simulink model "sistema4"  (R2026b)
settings: Solver=ode15s  MaxStep=1e-2
libraries: fl_lib x14, nesl_utility x6, slpidlib x1
settings Model: Creator=Admin  LastModifiedBy=nicol
settings DataIOCC: DSMLogging=off  ReturnWorkspaceOutputs=off  SaveOutput=off  SignalLogging=off  TimeSaveName=t
settings DebuggingCC: AlgebraicLoopMsg=none  ArtificialAlgebraicLoopMsg=none  MaxConsecutiveZCsMsg=none
settings RTWCC: GPUComputeCapability=5.0
settings SimscapeCC: SimscapeLogType=all  SimscapeNominalValues="[{\"value\":\"1\",\"unit\":\"A\"},{\"value\":\"1\",\"unit\":\"bar\"},{\"value\":\"1\",\"unit\":\"cm^2\"},{\"value\":\"1\",\"unit\":\"cm^3/s\"},{\"value\":\"1\",\"unit\":\"kJ/kg\"},{\"value\":\"1\",\"unit\":\"kW\"},{\"value\":\"1\",\"unit\":\"l\"},{\"value\":\"1\",\"unit\":\"N\"},{\"value\":\"1\",\"unit\":\"N*m\"},{\"value\":\"1\",\"unit\":\"V\"},{\"value\":\"0.001\",\"unit\":\"Wb\"}]"  SimscapeUseEnergyAccounting=off

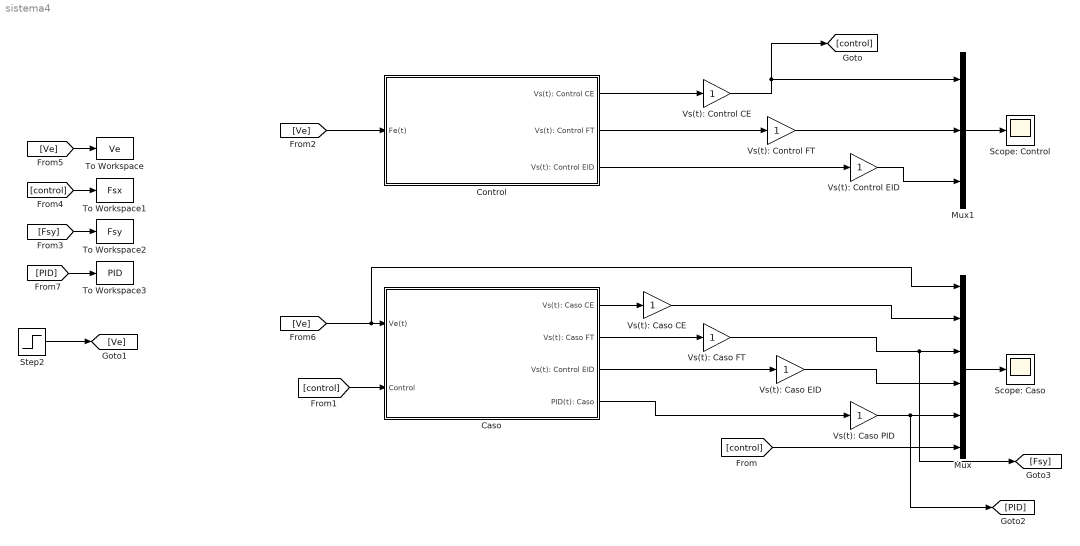
== system sistema4 ==
  Caso : Subsystem
  Control : Subsystem
  Mux : Mux  Inputs=6
  Mux1 : Mux  Inputs=3
  Scope: Caso : Scope
      settings: ActiveDisplayYMinimum=-0.12376521739333951  ActiveDisplayYMaximum=1.1138869565400558
  Scope: Control : Scope
      settings: ActiveDisplayYMinimum=-0.12376521739412114  ActiveDisplayYMaximum=1.1138869565470904
  Step2 : Step  Time=0  SampleTime=0
  To Workspace : ToWorkspace  VariableName=Ve  SampleTime=-1
  To Workspace1 : ToWorkspace  VariableName=Fsx  SampleTime=-1
  To Workspace2 : ToWorkspace  VariableName=Fsy  SampleTime=-1
  To Workspace3 : ToWorkspace  VariableName=PID  SampleTime=-1
  Vs(t): Caso CE : Gain
  Vs(t): Caso EID : Gain
  Vs(t): Caso FT : Gain
  Vs(t): Caso PID : Gain
  Vs(t): Control CE : Gain
  Vs(t): Control EID : Gain
  Vs(t): Control FT : Gain
  wires:
  Caso/2(Vs(t): Caso FT) -> Vs(t): Caso FT/1
  Caso/3(Vs(t): Control EID) -> Vs(t): Caso EID/1
  Vs(t): Caso EID/1 -> Mux/4
  Mux/1 -> Scope: Caso/1
  Mux1/1 -> Scope: Control/1
  Control/1(Vs(t): Control CE) -> Vs(t): Control CE/1
  [Ve] -> Control/1(Fe(t))
  [Ve] -> Mux/1, Caso/1(Ve(t))
  Control/3(Vs(t): Control EID) -> Vs(t): Control EID/1
  Vs(t): Control EID/1 -> Mux1/3
  Vs(t): Control FT/1 -> Mux1/2
  Control/2(Vs(t): Control FT) -> Vs(t): Control FT/1
  Caso/1(Vs(t): Caso CE) -> Vs(t): Caso CE/1
  Vs(t): Control CE/1 -> [control], Mux1/1
  Vs(t): Caso CE/1 -> Mux/2
  Vs(t): Caso FT/1 -> Mux/3, [Fsy]
  Caso/4(PID(t): Caso) -> Vs(t): Caso PID/1
  Vs(t): Caso PID/1 -> [PID], Mux/5
  [control] -> Mux/6
  [control] -> Caso/2(Control)
  [Fsy] -> To Workspace2/1
  [control] -> To Workspace1/1
  [PID] -> To Workspace3/1
  [Ve] -> To Workspace/1
  Step2/1 -> [Ve]

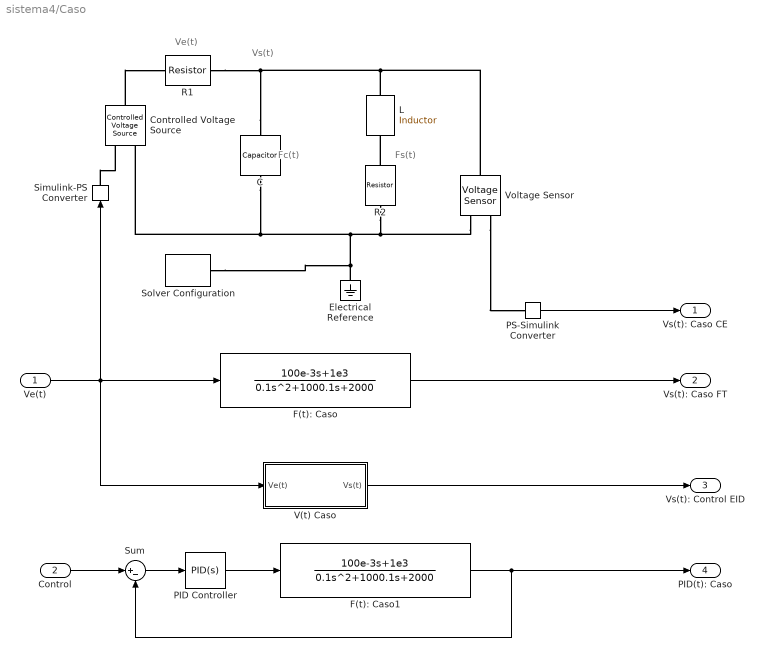
== system sistema4/Caso ==
  note: Ve(t)
  note: Vs(t)
  note: Fc(t)
  note: Fs(t)
  Ve(t) : Inport
  Control : Inport  Port=2
  C : fl_lib/Electrical/Electrical Elements/Capacitor  c=1000 uF  r=1e-6 Ohm  g=0 1/Ohm  i_specify=off  i_priority=None  i=0 A  i_nominal_specify=off  i_nominal_value=1  i_nominal_unit=A  v_specify=off  v_priority=None  v=0 V  v_nominal_specify=off  v_nominal_value=1  v_nominal_unit=V  vc_specify=off  vc_priority=High  vc=0 V  vc_nominal_specify=off  vc_nominal_value=1  vc_nominal_unit=V
  Controlled Voltage Source : fl_lib/Electrical/Electrical Sources/Controlled Voltage Source
  Electrical Reference : fl_lib/Electrical/Electrical Elements/Electrical Reference
  F(t): Caso : TransferFcn  Numerator=[100e-3 1e3]  Denominator=[0.1 1000.1 2000]
  F(t): Caso1 : TransferFcn  Numerator=[100e-3 1e3]  Denominator=[0.1 1000.1 2000]
  L : fl_lib/Electrical/Electrical Elements/Inductor  l=100e-3 H  r=0 Ohm  g=1e-9 1/Ohm  i_specify=off  i_priority=None  i=0 A  i_nominal_specify=off  i_nominal_value=1  i_nominal_unit=A  v_specify=off  v_priority=None  v=0 V  v_nominal_specify=off  v_nominal_value=1  v_nominal_unit=V  i_L_specify=off  i_L_priority=High  i_L=0 A  i_L_nominal_specify=off  i_L_nominal_value=1  i_L_nominal_unit=A
  PID Controller : slpidlib/PID Controller  Controller=PID  Form=Parallel  TimeDomain=Continuous-time  UseExternalTs=off  SampleTime=-1  IntegratorMethod=Forward Euler  FilterMethod=Forward Euler  ControllerParametersSource=internal  P=1315.96113707451  I=320705.002123674  UseKiTs=off  D=0.179701213263049  UseExternalDerivativeSource=off  N=5030.10216106345  UseFilter=on  TunerSelectOption=Transfer Function Based (PID Tuner App)  InitialConditionSource=internal  InitialConditionForIntegrator=0  InitialConditionForFilter=0  DifferentiatorICPrevScaledInput=0  ExternalReset=none  TrackingMode=off  Kt=1  LimitOutput=off  SatLimitsSource=internal  UpperSaturationLimit=inf  LowerSaturationLimit=-inf  LinearizeAsGain=on  AntiWindupMode=none  Kb=1  LimitIntegrator=off  UpperIntegratorSaturationLimit=inf  LowerIntegratorSaturationLimit=-inf  POutMin=[]  POutMax=[]  IOutMin=[]  IOutMax=[]  DOutMin=[]  DOutMax=[]  NOutMin=[]  NOutMax=[]  SumOutMin=[]  SumOutMax=[]  SaturationOutMin=[]  SaturationOutMax=[]  PParamMin=[]  PParamMax=[]  IParamMin=[]  IParamMax=[]  DParamMin=[]  DParamMax=[]  NParamMin=[]  NParamMax=[]  KbParamMin=[]  KbParamMax=[]  KtParamMin=[]  KtParamMax=[]  KbOutMin=[]  KbOutMax=[]  KtOutMin=[]  KtOutMax=[]  IntegratorOutMin=[]  IntegratorOutMax=[]  FilterOutMin=[]  FilterOutMax=[]  SumI1OutMin=[]  SumI1OutMax=[]  SumI2OutMin=[]  SumI2OutMax=[]  SumI3OutMin=[]  SumI3OutMax=[]  SumI4OutMin=[]  SumI4OutMax=[]  SumDOutMin=[]  SumDOutMax=[]  DifferentiatorOutMin=[]  DifferentiatorOutMax=[]  FilterDiffOutCoefMin=[]  FilterDiffOutCoefMax=[]  ReciprocalOutMin=[]  ReciprocalOutMax=[]  SumDenOutMin=[]  SumDenOutMax=[]  SumNumOutMin=[]  SumNumOutMax=[]  DivideOutMin=[]  DivideOutMax=[]  UdiffTsProdOutMin=[]  UdiffTsProdOutMax=[]  NTsProdOutMin=[]  NTsProdOutMax=[]  UintegralTsProdOutMin=[]  UintegralTsProdOutMax=[]  UngainTsProdOutMin=[]  UngainTsProdOutMax=[]  ClampingZeroOutDataTypeStr=Inherit: Inherit via back propagation  ClampingZeroOutMin=[]  ClampingZeroOutMax=[]  FilterDenConstantOutDataTypeStr=Inherit: Inherit via back propagation  FilterDenConstantOutMin=[]  FilterDenConstantOutMax=[]  PCopyOutDataTypeStr=Inherit: Inherit via back propagation  PCopyOutMin=[]  PCopyOutMax=[]  NCopyOutDataTypeStr=Inherit: Inherit via back propagation  NCopyOutMin=[]  NCopyOutMax=[]  IntegratorContinuousStateAttributes=''  IntegratorStateMustResolveToSignalObject=off  IntegratorRTWStateStorageClass=Auto  FilterContinuousStateAttributes=''  FilterStateMustResolveToSignalObject=off  FilterRTWStateStorageClass=Auto  ParallelPVariant=InternalParameters  IdealPVariant=Disabled  IVariant=InternalParameters  DVariant=InternalParameters  IntegratorVariant=Continuous  SatVariant=Disabled  AWVariant=Passthrough  PCopyVariant=Disabled  TRVariant=Disabled  FdbkBlocksVariant=Forward  IdealPFdbkVariant=Disabled  SatFdbkVariant=Disabled  DerivativeFilterVariant=ContFilter  NVariant=InternalParameters  NCopyVariant=Disabled  FilterICVariant=InternalICsFilter  IntegratorICVariant=InternalICs  ExternalResetVariant=Disabled  TRSumVariant=Passthrough  SumFdbkVariant=Disabled  SumVariant=Sum_PID  TsampFilterVariant=InternalTs  TsampNgainVariant=Passthrough  TsampIntegralVariant=Disabled_SignalSpec  ExternalSaturationOutDataTypeStr=Inherit: Same as second input  DerivativeSourceVariant=ErrorSignal  PreIntVariant=InternalPreInt
  PS-Simulink Converter : nesl_utility/PS-Simulink Converter  PhysicalDomain=network_engine_domain  SubClassName=ps_output  LeftPortType=input  RightPortType=output  PseudoPeriodic=off  Frequencies=[]  VectorFormat=inherit  Unit=inherit  AffineConversion=off
  R1 : fl_lib/Electrical/Electrical Elements/Resistor  R=1 kOhm  i_specify=off  i_priority=None  i=0 A  i_nominal_specify=off  i_nominal_value=1  i_nominal_unit=A  v_specify=off  v_priority=None  v=0 V  v_nominal_specify=off  v_nominal_value=1  v_nominal_unit=V
  R2 : fl_lib/Electrical/Electrical Elements/Resistor  R=1 kOhm  i_specify=off  i_priority=None  i=0 A  i_nominal_specify=off  i_nominal_value=1  i_nominal_unit=A  v_specify=off  v_priority=None  v=0 V  v_nominal_specify=off  v_nominal_value=1  v_nominal_unit=V
  Simulink-PS Converter : nesl_utility/Simulink-PS Converter  PhysicalDomain=network_engine_domain  SubClassName=ps_input  LeftPortType=input  RightPortType=output  PseudoPeriodic=off  Frequencies=[]  NoiseDistribution=none  NoiseParameters=[]  Unit=1  AffineConversion=off  FilteringAndDerivatives=provide  SimscapeFilterOrder=1  InputFilterTimeConstant=0.001  UdotUserProvided=0
  Solver Configuration : nesl_utility/Solver Configuration  PhysicalDomain=network_engine_domain  SubClassName=solver  LeftPortType=input  RightPortType=generic  Tones=[]  Harmonics=[]  SimulateNoise=off  Profile=off  UseLocalSampling=off  EnableSwitchedLinearOptims=on  FrequencyDomain=off  UseCCode=off  RelTol=0.001  AbsTol=0.001  MinStep=1e-09  ToWorkspace=off  RevertToSquareIcSolve=off  NumHomotopyIterations=100  PhasorMode=off  PhasorModeNumHarmonics=1  ConsistencySolver=NEWTON_XTOL_AFTER_FTOL  CanonicalOrdering=UNORDERED  OptimizeIntermediates=UNOPTIMIZED  MulticoreSolverChoice=BACKWARD_EULER  IndexReductionMethod=DerivativeReplacement  DoDC=off  ResidualTolerance=1e-09  ConsistencyTolSource=GLOBAL  ConsistencyAbsTol=0.001  ConsistencyRelTol=0.001  ConsistencyTolFactor=0.001  UseLocalSolver=off  LocalSolverChoice=NE_BACKWARD_EULER_ADVANCER  ResolveIndetEquations=on  FunctionEvalNumThread=1  LocalSolverSampleTime=0.001  DoFixedCost=off  MaxNonlinIter=3  MaxModeIter=2  ComputeImpulses=off  ImpulseIterations=2  LinearAlgebra=auto  LinearAlgebraNumThread=0  EquationFormulation=NE_TIME_EF  DelaysMemoryBudget=1024  AutomaticFiltering=on  FilteringTimeConstant=0.001  PartitionStorageMethod=AS_NEEDED  PartitionMemoryBudget=1024  PartitionMethod=BALANCED  MultibodyUseLocalSolver=off  MultibodyLocalSolverChoice=ODE1  MultibodyLocalSolverSampleTime=0.001
  Sum : Sum  Inputs=|+-
  V(t) Caso : Subsystem
  Voltage Sensor : fl_lib/Electrical/Electrical Sensors/Voltage Sensor
  Vs(t): Caso CE : Outport
  Vs(t): Caso FT : Outport  Port=2
  Vs(t): Control EID : Outport  Port=3
  PID(t): Caso : Outport  Port=4
  wires:
  Ve(t)/1 -> V(t) Caso/1(Ve(t)), F(t): Caso/1, Simulink-PS Converter/1
  PS-Simulink Converter/1 -> Vs(t): Caso CE/1
  F(t): Caso/1 -> Vs(t): Caso FT/1
  V(t) Caso/1(Vs(t)) -> Vs(t): Control EID/1
  PID Controller/1 -> F(t): Caso1/1
  F(t): Caso1/1 -> Sum/2, PID(t): Caso/1
  Sum/1 -> PID Controller/1
  Control/1 -> Sum/1
  connections:
  Simulink-PS Converter/RConn1 -- Controlled Voltage Source/RConn1
  Controlled Voltage Source/RConn2 -- C/RConn1 -- Solver Configuration/RConn1 -- Electrical Reference/LConn1 -- R2/LConn1 -- Voltage Sensor/RConn2
  Controlled Voltage Source/LConn1 -- R1/RConn1
  C/LConn1 -- R1/LConn1 -- L/LConn1 -- Voltage Sensor/LConn1
  R2/RConn1 -- L/RConn1
  Voltage Sensor/RConn1 -- PS-Simulink Converter/LConn1

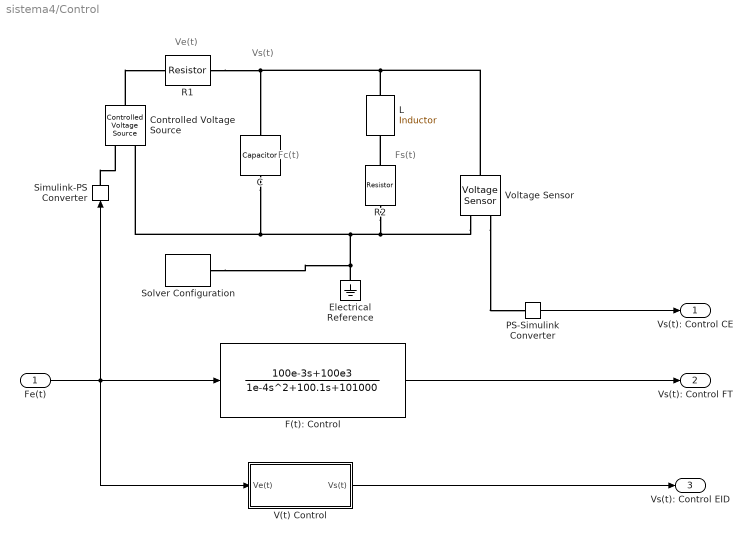
== system sistema4/Control ==
  note: Ve(t)
  note: Vs(t)
  note: Fc(t)
  note: Fs(t)
  Fe(t) : Inport
  C : fl_lib/Electrical/Electrical Elements/Capacitor  c=1 uF  r=1e-6 Ohm  g=0 1/Ohm  i_specify=off  i_priority=None  i=0 A  i_nominal_specify=off  i_nominal_value=1  i_nominal_unit=A  v_specify=off  v_priority=None  v=0 V  v_nominal_specify=off  v_nominal_value=1  v_nominal_unit=V  vc_specify=off  vc_priority=High  vc=0 V  vc_nominal_specify=off  vc_nominal_value=1  vc_nominal_unit=V
  Controlled Voltage Source : fl_lib/Electrical/Electrical Sources/Controlled Voltage Source
  Electrical Reference : fl_lib/Electrical/Electrical Elements/Electrical Reference
  F(t): Control : TransferFcn  Numerator=[100e-3 100e3]  Denominator=[1e-4 100.1 101000]
  L : fl_lib/Electrical/Electrical Elements/Inductor  l=100e-3 H  r=0 Ohm  g=1e-9 1/Ohm  i_specify=off  i_priority=None  i=0 A  i_nominal_specify=off  i_nominal_value=1  i_nominal_unit=A  v_specify=off  v_priority=None  v=0 V  v_nominal_specify=off  v_nominal_value=1  v_nominal_unit=V  i_L_specify=off  i_L_priority=High  i_L=0 A  i_L_nominal_specify=off  i_L_nominal_value=1  i_L_nominal_unit=A
  PS-Simulink Converter : nesl_utility/PS-Simulink Converter  PhysicalDomain=network_engine_domain  SubClassName=ps_output  LeftPortType=input  RightPortType=output  PseudoPeriodic=off  Frequencies=[]  VectorFormat=inherit  Unit=inherit  AffineConversion=off
  R1 : fl_lib/Electrical/Electrical Elements/Resistor  R=1 kOhm  i_specify=off  i_priority=None  i=0 A  i_nominal_specify=off  i_nominal_value=1  i_nominal_unit=A  v_specify=off  v_priority=None  v=0 V  v_nominal_specify=off  v_nominal_value=1  v_nominal_unit=V
  R2 : fl_lib/Electrical/Electrical Elements/Resistor  R=100 kOhm  i_specify=off  i_priority=None  i=0 A  i_nominal_specify=off  i_nominal_value=1  i_nominal_unit=A  v_specify=off  v_priority=None  v=0 V  v_nominal_specify=off  v_nominal_value=1  v_nominal_unit=V
  Simulink-PS Converter : nesl_utility/Simulink-PS Converter  PhysicalDomain=network_engine_domain  SubClassName=ps_input  LeftPortType=input  RightPortType=output  PseudoPeriodic=off  Frequencies=[]  NoiseDistribution=none  NoiseParameters=[]  Unit=1  AffineConversion=off  FilteringAndDerivatives=provide  SimscapeFilterOrder=1  InputFilterTimeConstant=0.001  UdotUserProvided=0
  Solver Configuration : nesl_utility/Solver Configuration  PhysicalDomain=network_engine_domain  SubClassName=solver  LeftPortType=input  RightPortType=generic  Tones=[]  Harmonics=[]  SimulateNoise=off  Profile=off  UseLocalSampling=off  EnableSwitchedLinearOptims=on  FrequencyDomain=off  UseCCode=off  RelTol=0.001  AbsTol=0.001  MinStep=1e-09  ToWorkspace=off  RevertToSquareIcSolve=off  NumHomotopyIterations=100  PhasorMode=off  PhasorModeNumHarmonics=1  ConsistencySolver=NEWTON_XTOL_AFTER_FTOL  CanonicalOrdering=UNORDERED  OptimizeIntermediates=UNOPTIMIZED  MulticoreSolverChoice=BACKWARD_EULER  IndexReductionMethod=DerivativeReplacement  DoDC=off  ResidualTolerance=1e-09  ConsistencyTolSource=GLOBAL  ConsistencyAbsTol=0.001  ConsistencyRelTol=0.001  ConsistencyTolFactor=0.001  UseLocalSolver=off  LocalSolverChoice=NE_BACKWARD_EULER_ADVANCER  ResolveIndetEquations=on  FunctionEvalNumThread=1  LocalSolverSampleTime=0.001  DoFixedCost=off  MaxNonlinIter=3  MaxModeIter=2  ComputeImpulses=off  ImpulseIterations=2  LinearAlgebra=auto  LinearAlgebraNumThread=0  EquationFormulation=NE_TIME_EF  DelaysMemoryBudget=1024  AutomaticFiltering=on  FilteringTimeConstant=0.001  PartitionStorageMethod=AS_NEEDED  PartitionMemoryBudget=1024  PartitionMethod=BALANCED  MultibodyUseLocalSolver=off  MultibodyLocalSolverChoice=ODE1  MultibodyLocalSolverSampleTime=0.001
  V(t) Control : Subsystem
  Voltage Sensor : fl_lib/Electrical/Electrical Sensors/Voltage Sensor
  Vs(t): Control CE : Outport
  Vs(t): Control FT : Outport  Port=2
  Vs(t): Control EID : Outport  Port=3
  wires:
  Fe(t)/1 -> V(t) Control/1(Ve(t)), F(t): Control/1, Simulink-PS Converter/1
  PS-Simulink Converter/1 -> Vs(t): Control CE/1
  F(t): Control/1 -> Vs(t): Control FT/1
  V(t) Control/1(Vs(t)) -> Vs(t): Control EID/1
  connections:
  Simulink-PS Converter/RConn1 -- Controlled Voltage Source/RConn1
  Solver Configuration/RConn1 -- Electrical Reference/LConn1 -- Voltage Sensor/RConn2 -- R2/LConn1 -- Controlled Voltage Source/RConn2 -- C/RConn1
  Controlled Voltage Source/LConn1 -- R1/RConn1
  R1/LConn1 -- Voltage Sensor/LConn1 -- L/LConn1 -- C/LConn1
  R2/RConn1 -- L/RConn1
  Voltage Sensor/RConn1 -- PS-Simulink Converter/LConn1

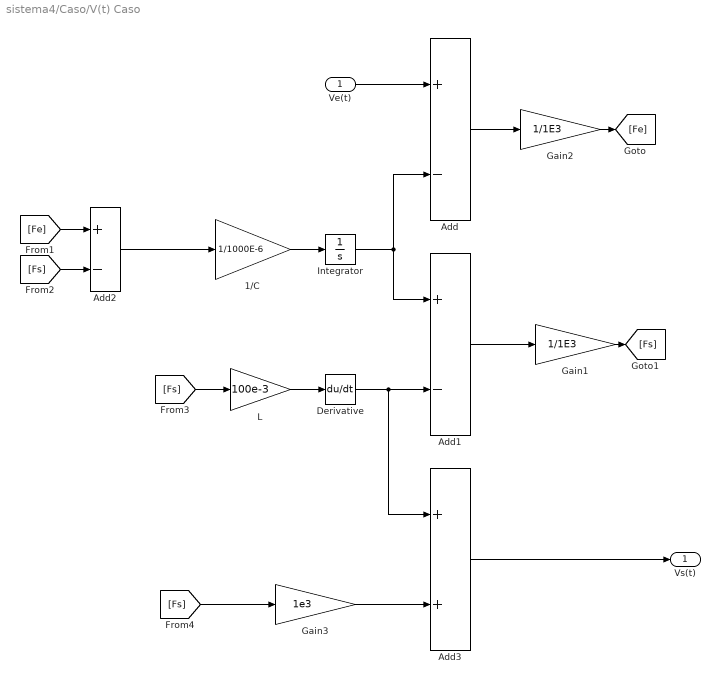
== system sistema4/Caso/V(t) Caso ==
  Ve(t) : Inport
  1/C : Gain  Gain=1/1000E-6
  Add : Sum  Inputs=+-
  Add1 : Sum  Inputs=+-
  Add2 : Sum  Inputs=+-
  Add3 : Sum
  Derivative : Derivative
  Gain1 : Gain  Gain=1/1E3
  Gain2 : Gain  Gain=1/1E3
  Gain3 : Gain  Gain=1e3
  Integrator : Integrator
  L : Gain  Gain=100e-3
  Vs(t) : Outport
  wires:
  [Fe] -> Add2/1
  Add1/1 -> Gain1/1
  Ve(t)/1 -> Add/1
  [Fs] -> Add2/2
  Add/1 -> Gain2/1
  Gain2/1 -> [Fe]
  Gain1/1 -> [Fs]
  1/C/1 -> Integrator/1
  Integrator/1 -> Add1/1, Add/2
  Add2/1 -> 1/C/1
  Derivative/1 -> Add3/1, Add1/2
  L/1 -> Derivative/1
  [Fs] -> L/1
  [Fs] -> Gain3/1
  Gain3/1 -> Add3/2
  Add3/1 -> Vs(t)/1

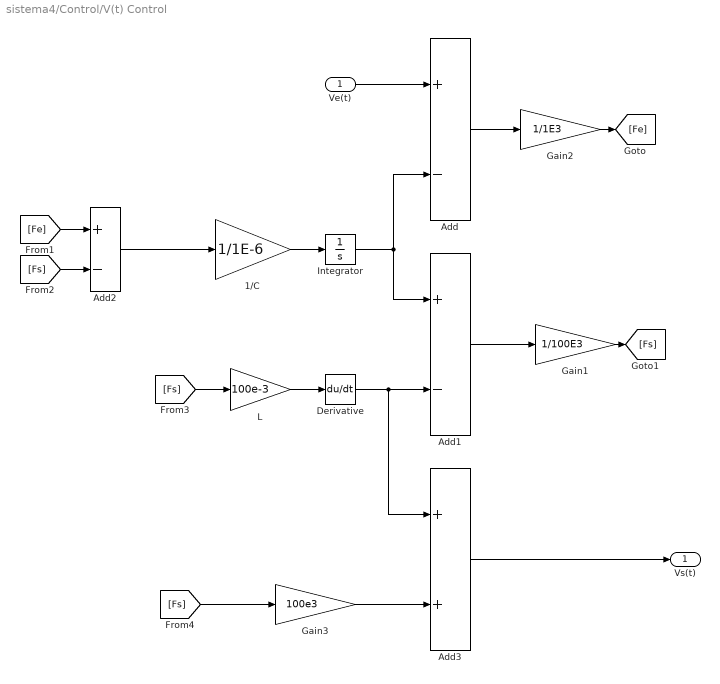
== system sistema4/Control/V(t) Control ==
  Ve(t) : Inport
  1/C : Gain  Gain=1/1E-6
  Add : Sum  Inputs=+-
  Add1 : Sum  Inputs=+-
  Add2 : Sum  Inputs=+-
  Add3 : Sum
  Derivative : Derivative
  Gain1 : Gain  Gain=1/100E3
  Gain2 : Gain  Gain=1/1E3
  Gain3 : Gain  Gain=100e3
  Integrator : Integrator
  L : Gain  Gain=100e-3
  Vs(t) : Outport
  wires:
  [Fe] -> Add2/1
  Add1/1 -> Gain1/1
  Ve(t)/1 -> Add/1
  [Fs] -> Add2/2
  Add/1 -> Gain2/1
  Gain2/1 -> [Fe]
  Gain1/1 -> [Fs]
  1/C/1 -> Integrator/1
  Integrator/1 -> Add1/1, Add/2
  Add2/1 -> 1/C/1
  Derivative/1 -> Add3/1, Add1/2
  L/1 -> Derivative/1
  [Fs] -> L/1
  [Fs] -> Gain3/1
  Gain3/1 -> Add3/2
  Add3/1 -> Vs(t)/1
